simulink model "cs_rectifier_average"  (R2026a)
settings: Solver=ode15s  StopTime=460  MaxStep=0.01  RelTol=1e-6
model workspace (MAT data in the model file):
  B_base = 13
  I_base = 45000
  Ki_vdc_alpha = 0.2
  Kp_vdc_alpha = 0.005
  LGrid = [1.1 1.09999989603 1.09999958429 1.09999906509 1.09999833871 1.09999740544 1.09999626556 1.09999491937 1.09999336715 1.09999160919 1.09998964578 1.09998747721 ... (46001 elements, 1x46001)]
  LKey = [1.1 1.08 1.03 0.98 0.95 1.02 1 1.08 1.12]
  L_ts : timeseries (value not decoded)
  RGrid = [0.35 0.351877050317 0.3537498692 0.35561845855 0.357482820267 0.35934295625 0.3611988684 0.363050558617 0.3648980288 0.36674128085 0.368580316667 0.37041513815 ... (46001 elements, 1x46001)]
  RKey = [0.35 0.8 0.6 0.024 0.024 0.12 0.12 0.25 0.35]
  R_ts : timeseries (value not decoded)
  S_transformer = 70000000
  V_primary = 10000
  V_secondary = 1200
  Vdc_filter_a = 0.995012479193
  Vdc_filter_tau = 0.01
  Vdc_ref = 1500
  alpha0_deg = 22.1916065663
  alpha_integral_max = 57.8083934337
  alpha_integral_min = -17.1916065663
  alpha_max_deg = 80
  alpha_min_deg = 5
  avg_Ki_deg_per_Vs = 0.5
  avg_Kp_deg_per_V = 0.02
  avg_converter_tau_s = 0.05
  control_sample_time = 5e-05
  dt = 0.01
  kB = 0.000288888888889
  tGrid = [0 0.01 0.02 0.03 0.04 0.05 0.06 0.07 0.08 0.09 0.1 0.11 ... (46001 elements, 1x46001)]
  tKey = [0 5 8 12 45 70 335 420 460]
  transformer_ratio = 0.12
libraries: nesl_utility x6, fl_lib x5, ee_lib x1
(part 2 of 2)

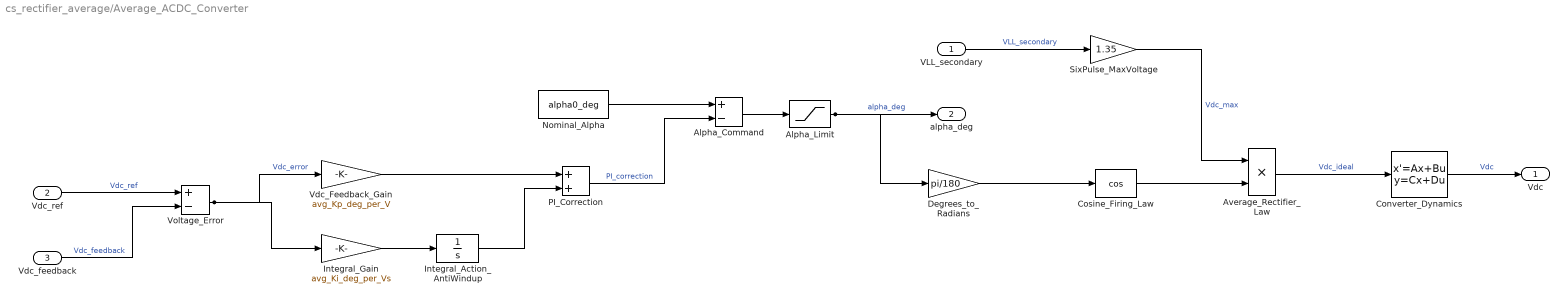
== system cs_rectifier_average/Average_ACDC_Converter ==
  VLL_secondary : Inport
  Vdc_ref : Inport  Port=2
  Vdc_feedback : Inport  Port=3
  Alpha_Command : Sum  Inputs=+-
  Alpha_Limit : Saturate  UpperLimit=80  LowerLimit=5
  Average_Rectifier_Law : Product  Inputs=**
  Converter_Dynamics : StateSpace  A=-1/avg_converter_tau_s  B=1/avg_converter_tau_s  D=0  InitialCondition=Vdc_ref
  Cosine_Firing_Law : Trigonometry  Operator=cos
  Degrees_to_Radians : Gain  Gain=pi/180
  Integral_Action_AntiWindup : Integrator  LimitOutput=on  UpperSaturationLimit=20  LowerSaturationLimit=-60
  Integral_Gain : Gain  Gain=avg_Ki_deg_per_Vs
  Nominal_Alpha : Constant  Value=alpha0_deg
  PI_Correction : Sum
  SixPulse_MaxVoltage : Gain  Gain=1.35
  Vdc_Feedback_Gain : Gain  Gain=avg_Kp_deg_per_V
  Voltage_Error : Sum  Inputs=+-
  Vdc : Outport
  alpha_deg : Outport  Port=2
  wires:
  PI_Correction/1 -> Alpha_Command/2  "PI_correction"
  Integral_Action_AntiWindup/1 -> PI_Correction/2
  Vdc_Feedback_Gain/1 -> PI_Correction/1
  Integral_Gain/1 -> Integral_Action_AntiWindup/1
  Vdc_ref/1 -> Voltage_Error/1  "Vdc_ref"
  Vdc_feedback/1 -> Voltage_Error/2  "Vdc_feedback"
  Voltage_Error/1 -> Integral_Gain/1, Vdc_Feedback_Gain/1  "Vdc_error"
  Nominal_Alpha/1 -> Alpha_Command/1
  Alpha_Command/1 -> Alpha_Limit/1
  Alpha_Limit/1 -> Degrees_to_Radians/1, alpha_deg/1  "alpha_deg"
  Degrees_to_Radians/1 -> Cosine_Firing_Law/1
  VLL_secondary/1 -> SixPulse_MaxVoltage/1  "VLL_secondary"
  SixPulse_MaxVoltage/1 -> Average_Rectifier_Law/1  "Vdc_max"
  Cosine_Firing_Law/1 -> Average_Rectifier_Law/2
  Average_Rectifier_Law/1 -> Converter_Dynamics/1  "Vdc_ideal"
  Converter_Dynamics/1 -> Vdc/1  "Vdc"

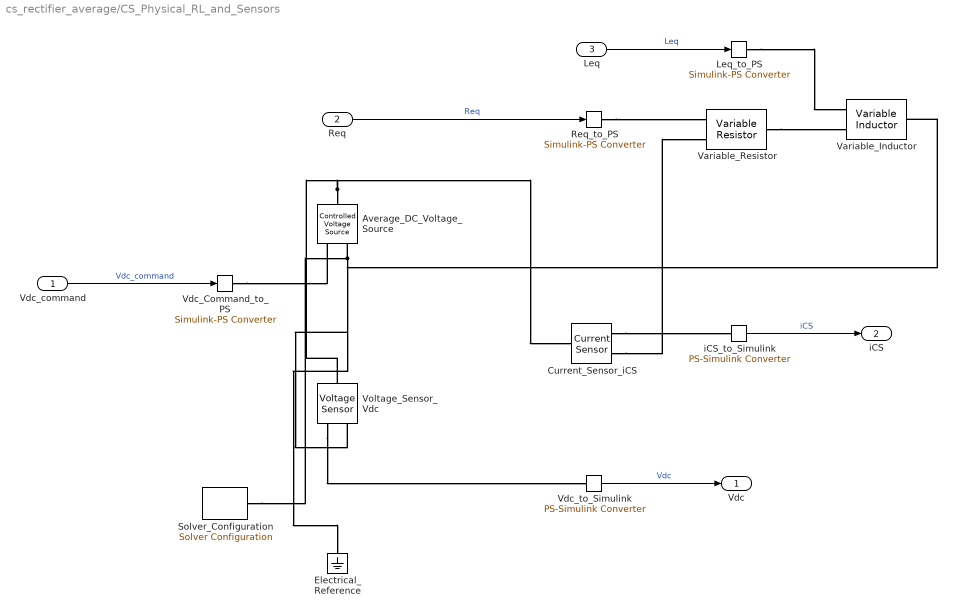
== system cs_rectifier_average/CS_Physical_RL_and_Sensors ==
  Vdc_command : Inport
  Req : Inport  Port=2
  Leq : Inport  Port=3
  Average_DC_Voltage_Source : fl_lib/Electrical/Electrical Sources/Controlled Voltage Source
  Current_Sensor_iCS : fl_lib/Electrical/Electrical Sensors/Current Sensor
  Electrical_Reference : fl_lib/Electrical/Electrical Elements/Electrical Reference
  Leq_to_PS : nesl_utility/Simulink-PS Converter  PhysicalDomain=network_engine_domain  SubClassName=ps_input  LeftPortType=input  RightPortType=output  PseudoPeriodic=off  Frequencies=[]  NoiseDistribution=none  NoiseParameters=[]  Unit=H  AffineConversion=off  FilteringAndDerivatives=provide  SimscapeFilterOrder=1  InputFilterTimeConstant=0.001  UdotUserProvided=0
  Req_to_PS : nesl_utility/Simulink-PS Converter  PhysicalDomain=network_engine_domain  SubClassName=ps_input  LeftPortType=input  RightPortType=output  PseudoPeriodic=off  Frequencies=[]  NoiseDistribution=none  NoiseParameters=[]  Unit=Ohm  AffineConversion=off  FilteringAndDerivatives=provide  SimscapeFilterOrder=1  InputFilterTimeConstant=0.001  UdotUserProvided=0
  Solver_Configuration : nesl_utility/Solver Configuration  PhysicalDomain=network_engine_domain  SubClassName=solver  LeftPortType=input  RightPortType=generic  Tones=[]  Harmonics=[]  SimulateNoise=off  Profile=off  UseLocalSampling=off  EnableSwitchedLinearOptims=on  FrequencyDomain=off  UseCCode=off  RelTol=0.001  AbsTol=0.001  MinStep=1e-09  ToWorkspace=off  RevertToSquareIcSolve=off  NumHomotopyIterations=100  PhasorMode=off  PhasorModeNumHarmonics=1  ConsistencySolver=NEWTON_XTOL_AFTER_FTOL  CanonicalOrdering=UNORDERED  OptimizeIntermediates=UNOPTIMIZED  IndexReductionMethod=DerivativeReplacement  DoDC=off  ResidualTolerance=1e-09  ConsistencyTolSource=GLOBAL  ConsistencyAbsTol=0.001  ConsistencyRelTol=0.001  ConsistencyTolFactor=0.001  UseLocalSolver=off  LocalSolverChoice=NE_BACKWARD_EULER_ADVANCER  ResolveIndetEquations=on  FunctionEvalNumThread=1  LocalSolverSampleTime=0.001  DoFixedCost=off  MaxNonlinIter=3  MaxModeIter=2  ComputeImpulses=off  ImpulseIterations=2  LinearAlgebra=auto  LinearAlgebraNumThread=0  EquationFormulation=NE_TIME_EF  DelaysMemoryBudget=1024  AutomaticFiltering=on  FilteringTimeConstant=0.001  PartitionStorageMethod=AS_NEEDED  PartitionMemoryBudget=1024  PartitionMethod=ROBUST  MultibodyUseLocalSolver=off  MultibodyLocalSolverChoice=ODE1  MultibodyLocalSolverSampleTime=0.001
  Variable_Inductor : ee_lib/Passive/Variable Inductor  prm=1  Lmin=1e-3 H  g=1e-9 1/Ohm  i0=0 A  phi0=0 Wb
  Variable_Resistor : fl_lib/Electrical/Electrical Elements/Variable Resistor  Rmin=1e-4 Ohm  thermalEnable=false  thermal_mass=1 J/K  i_specify=off  i_priority=None  i=0 A  i_nominal_specify=off  i_nominal_value=1  i_nominal_unit=A  v_specify=off  v_priority=None  v=0 V  v_nominal_specify=off  v_nominal_value=1  v_nominal_unit=V  T_specify=off  T_priority=None  T=300 K  T_nominal_specify=off  T_nominal_value=1  T_nominal_unit=K
  Vdc_Command_to_PS : nesl_utility/Simulink-PS Converter  PhysicalDomain=network_engine_domain  SubClassName=ps_input  LeftPortType=input  RightPortType=output  PseudoPeriodic=off  Frequencies=[]  NoiseDistribution=none  NoiseParameters=[]  Unit=V  AffineConversion=off  FilteringAndDerivatives=provide  SimscapeFilterOrder=1  InputFilterTimeConstant=0.001  UdotUserProvided=0
  Vdc_to_Simulink : nesl_utility/PS-Simulink Converter  PhysicalDomain=network_engine_domain  SubClassName=ps_output  LeftPortType=input  RightPortType=output  PseudoPeriodic=off  Frequencies=[]  VectorFormat=inherit  Unit=V  AffineConversion=off
  Voltage_Sensor_Vdc : fl_lib/Electrical/Electrical Sensors/Voltage Sensor
  iCS_to_Simulink : nesl_utility/PS-Simulink Converter  PhysicalDomain=network_engine_domain  SubClassName=ps_output  LeftPortType=input  RightPortType=output  PseudoPeriodic=off  Frequencies=[]  VectorFormat=inherit  Unit=A  AffineConversion=off
  Vdc : Outport
  iCS : Outport  Port=2
  wires:
  iCS_to_Simulink/1 -> iCS/1  "iCS"
  Vdc_to_Simulink/1 -> Vdc/1  "Vdc"
  Leq/1 -> Leq_to_PS/1  "Leq"
  Req/1 -> Req_to_PS/1  "Req"
  Vdc_command/1 -> Vdc_Command_to_PS/1  "Vdc_command"
  connections:
  Current_Sensor_iCS/RConn1 -- iCS_to_Simulink/LConn1
  Voltage_Sensor_Vdc/RConn1 -- Vdc_to_Simulink/LConn1
  Average_DC_Voltage_Source/RConn2 -- Solver_Configuration/RConn1 -- Electrical_Reference/LConn1 -- Voltage_Sensor_Vdc/RConn2 -- Variable_Inductor/RConn1
  Variable_Resistor/RConn1 -- Variable_Inductor/LConn2
  Current_Sensor_iCS/RConn2 -- Variable_Resistor/LConn2
  Average_DC_Voltage_Source/LConn1 -- Voltage_Sensor_Vdc/LConn1 -- Current_Sensor_iCS/LConn1
  Leq_to_PS/RConn1 -- Variable_Inductor/LConn1
  Req_to_PS/RConn1 -- Variable_Resistor/LConn1
  Vdc_Command_to_PS/RConn1 -- Average_DC_Voltage_Source/RConn1

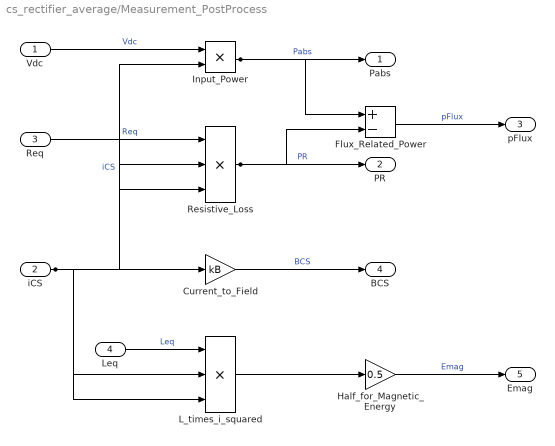
== system cs_rectifier_average/Measurement_PostProcess ==
  Vdc : Inport
  iCS : Inport  Port=2
  Req : Inport  Port=3
  Leq : Inport  Port=4
  Current_to_Field : Gain  Gain=kB
  Flux_Related_Power : Sum  Inputs=+-
  Half_for_Magnetic_Energy : Gain  Gain=0.5
  Input_Power : Product  Inputs=**
  L_times_i_squared : Product  Inputs=***
  Resistive_Loss : Product  Inputs=***
  Pabs : Outport
  PR : Outport  Port=2
  pFlux : Outport  Port=3
  BCS : Outport  Port=4
  Emag : Outport  Port=5
  wires:
  Half_for_Magnetic_Energy/1 -> Emag/1  "Emag"
  L_times_i_squared/1 -> Half_for_Magnetic_Energy/1
  Leq/1 -> L_times_i_squared/1  "Leq"
  Current_to_Field/1 -> BCS/1  "BCS"
  Flux_Related_Power/1 -> pFlux/1  "pFlux"
  Req/1 -> Resistive_Loss/1  "Req"
  iCS/1 -> L_times_i_squared/3, L_times_i_squared/2, Current_to_Field/1, Resistive_Loss/3, Resistive_Loss/2, Input_Power/2  "iCS"
  Vdc/1 -> Input_Power/1  "Vdc"
  Input_Power/1 -> Pabs/1, Flux_Related_Power/1  "Pabs"
  Resistive_Loss/1 -> PR/1, Flux_Related_Power/2  "PR"

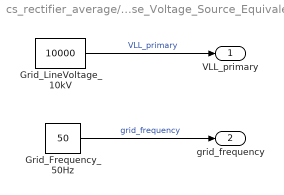
== system cs_rectifier_average/Three_Phase_Voltage_Source_Equivalent ==
  Grid_Frequency_50Hz : Constant  Value=50
  Grid_LineVoltage_10kV : Constant  Value=10000
  VLL_primary : Outport
  grid_frequency : Outport  Port=2
  wires:
  Grid_LineVoltage_10kV/1 -> VLL_primary/1  "VLL_primary"
  Grid_Frequency_50Hz/1 -> grid_frequency/1  "grid_frequency"

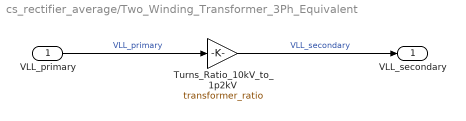
== system cs_rectifier_average/Two_Winding_Transformer_3Ph_Equivalent ==
  VLL_primary : Inport
  Turns_Ratio_10kV_to_1p2kV : Gain  Gain=transformer_ratio
  VLL_secondary : Outport
  wires:
  Turns_Ratio_10kV_to_1p2kV/1 -> VLL_secondary/1  "VLL_secondary"
  VLL_primary/1 -> Turns_Ratio_10kV_to_1p2kV/1  "VLL_primary"
